simulink model "LithiumIonSieve"  (R2025b)
settings: Solver=VariableStepAuto  StartTime=0.0  StopTime=3600*48  RelTol=1e-3
undefined symbols (not defined in the file or in its folder): t_clean, t_regen, t_service
libraries: fl_lib x19, customization_lib x14, nesl_utility x1
settings Model: Creator=ndegoede  LastModifiedBy=degoede
settings SimscapeCC: SimscapeLogType=all  SimscapeLogOpenViewer=on

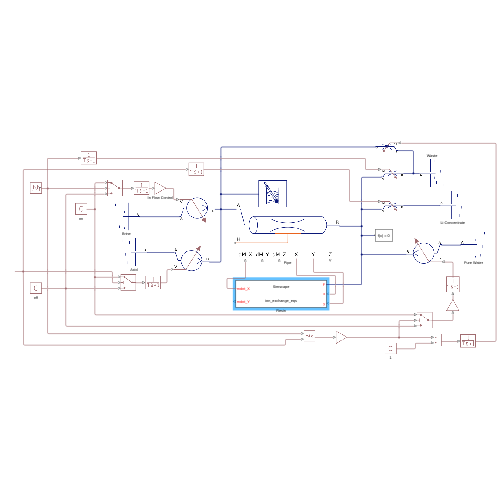
[thumbnail: Simulink's stored preview of the top-level diagram]
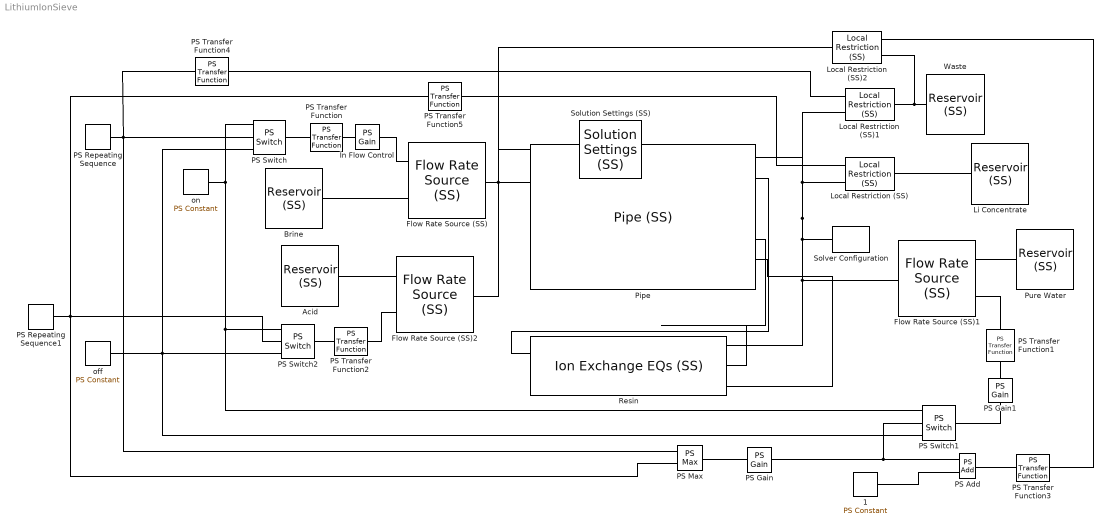
== system LithiumIonSieve ==
  1 : fl_lib/Physical Signals/Sources/PS Constant  constant=1
  Acid : customization_lib/solution/elements/Reservoir (SS)  pressure_spec=foundation.enum.pressure_spec.atmospheric  reservoir_pressure=0.101325 MPa  reservoir_temperature=293.15 K  reservoir_concentration=0 kg/m^3  reservoir_concentration_y=2e-4 g/l  reservoir_concentration_z=0 kg/m^3  area=0.01 m^2  custom_ports=false  length_A=1e-3 m
      settings: SourceProductName=Customization  InternalSimscapePortConfiguration="{\"Bottom\":[],\"Left\":[{\"id\":\"A\",\"label\":\"A\",\"type\":\"customization.solution.solution\"}],\"Right\":[],\"Top\":[]}"
  Brine : customization_lib/solution/elements/Reservoir (SS)  pressure_spec=foundation.enum.pressure_spec.atmospheric  reservoir_pressure=0.101325 MPa  reservoir_temperature=293.15 K  reservoir_concentration=1630 mg/l  reservoir_concentration_y=10^-6.5 g/l  reservoir_concentration_z=29000 mg/l  area=0.01 m^2  custom_ports=false  length_A=1e-3 m
      settings: SourceProductName=Customization  InternalSimscapePortConfiguration="{\"Bottom\":[],\"Left\":[{\"id\":\"A\",\"label\":\"A\",\"type\":\"customization.solution.solution\"}],\"Right\":[],\"Top\":[]}"
  Flow Rate Source (SS) : customization_lib/solution/sources/Flow Rate Source (SS)  source_type=foundation.enum.constant_controlled.controlled  flow_type=foundation.enum.mass_volumetric_flow.volumetric  mass_flow=0 kg/s  volumetric_flow=0 m^3/s  power_spec=foundation.enum.power_spec.isentropic  area=0.01 m^2  custom_ports=false  length_A=1e-3 m  length_B=1e-3 m
      settings: SourceProductName=Customization  InternalSimscapePortConfiguration="{\"Bottom\":[],\"Left\":[{\"id\":\"A\",\"label\":\"A\",\"type\":\"customization.solution.solution\"},{\"id\":\"V\",\"label\":\"V\",\"type\":\"input\"}],\"Right\":[{\"id\":\"B\",\"label\":\"B\",\"type\":\"customization.solution.solution\"}],\"Top\":[]}"
  Flow Rate Source (SS)1 : customization_lib/solution/sources/Flow Rate Source (SS)  source_type=foundation.enum.constant_controlled.controlled  flow_type=foundation.enum.mass_volumetric_flow.volumetric  mass_flow=0 kg/s  volumetric_flow=0 m^3/s  power_spec=foundation.enum.power_spec.isentropic  area=0.01 m^2  custom_ports=false  length_A=1e-3 m  length_B=1e-3 m
      settings: SourceProductName=Customization  InternalSimscapePortConfiguration="{\"Bottom\":[],\"Left\":[{\"id\":\"A\",\"label\":\"A\",\"type\":\"customization.solution.solution\"},{\"id\":\"V\",\"label\":\"V\",\"type\":\"input\"}],\"Right\":[{\"id\":\"B\",\"label\":\"B\",\"type\":\"customization.solution.solution\"}],\"Top\":[]}"
  Flow Rate Source (SS)2 : customization_lib/solution/sources/Flow Rate Source (SS)  source_type=foundation.enum.constant_controlled.controlled  flow_type=foundation.enum.mass_volumetric_flow.volumetric  mass_flow=0 kg/s  volumetric_flow=0 m^3/s  power_spec=foundation.enum.power_spec.isentropic  area=0.01 m^2  custom_ports=false  length_A=1e-3 m  length_B=1e-3 m
      settings: SourceProductName=Customization  InternalSimscapePortConfiguration="{\"Bottom\":[],\"Left\":[{\"id\":\"A\",\"label\":\"A\",\"type\":\"customization.solution.solution\"},{\"id\":\"V\",\"label\":\"V\",\"type\":\"input\"}],\"Right\":[{\"id\":\"B\",\"label\":\"B\",\"type\":\"customization.solution.solution\"}],\"Top\":[]}"
  In Flow Control : fl_lib/Physical Signals/Functions/PS Gain  gain=2
  Li Concentrate : customization_lib/solution/elements/Reservoir (SS)  pressure_spec=foundation.enum.pressure_spec.atmospheric  reservoir_pressure=0.101325 MPa  reservoir_temperature=293.15 K  reservoir_concentration=0 kg/m^3  reservoir_concentration_y=0 kg/m^3  reservoir_concentration_z=0 kg/m^3  area=0.01 m^2  custom_ports=false  length_A=1e-3 m
      settings: SourceProductName=Customization  InternalSimscapePortConfiguration="{\"Bottom\":[],\"Left\":[{\"id\":\"A\",\"label\":\"A\",\"type\":\"customization.solution.solution\"}],\"Right\":[],\"Top\":[]}"
  Local Restriction (SS) : customization_lib/solution/elements/Local Restriction (SS)  restriction_type=foundation.enum.restriction_type.variable  restriction_area=0.001 m^2  min_area=1e-5 m^2  max_area=0.005 m^2  area=0.01 m^2  Cd=0.64  Re_c=150  pressure_recovery=simscape.enum.onoff.on  custom_ports=false  length_A=1e-3 m  length_B=1e-3 m
      settings: SourceProductName=Customization  InternalSimscapePortConfiguration="{\"Bottom\":[],\"Left\":[{\"id\":\"A\",\"label\":\"A\",\"type\":\"customization.solution.solution\"},{\"id\":\"area_in\",\"label\":\"AR\",\"type\":\"input\"}],\"Right\":[{\"id\":\"B\",\"label\":\"B\",\"type\":\"customization.solution.solution\"}],\"Top\":[]}"
  Local Restriction (SS)1 : customization_lib/solution/elements/Local Restriction (SS)  restriction_type=foundation.enum.restriction_type.variable  restriction_area=0.001 m^2  min_area=1e-5 m^2  max_area=0.005 m^2  area=0.01 m^2  Cd=0.64  Re_c=150  pressure_recovery=simscape.enum.onoff.on  custom_ports=false  length_A=1e-3 m  length_B=1e-3 m
      settings: SourceProductName=Customization  InternalSimscapePortConfiguration="{\"Bottom\":[],\"Left\":[{\"id\":\"A\",\"label\":\"A\",\"type\":\"customization.solution.solution\"},{\"id\":\"area_in\",\"label\":\"AR\",\"type\":\"input\"}],\"Right\":[{\"id\":\"B\",\"label\":\"B\",\"type\":\"customization.solution.solution\"}],\"Top\":[]}"
  Local Restriction (SS)2 : customization_lib/solution/elements/Local Restriction (SS)  restriction_type=foundation.enum.restriction_type.variable  restriction_area=0.001 m^2  min_area=1e-5 m^2  max_area=0.005 m^2  area=0.01 m^2  Cd=0.64  Re_c=150  pressure_recovery=simscape.enum.onoff.on  custom_ports=false  length_A=1e-3 m  length_B=1e-3 m
      settings: SourceProductName=Customization  InternalSimscapePortConfiguration="{\"Bottom\":[],\"Left\":[{\"id\":\"A\",\"label\":\"A\",\"type\":\"customization.solution.solution\"},{\"id\":\"area_in\",\"label\":\"AR\",\"type\":\"input\"}],\"Right\":[{\"id\":\"B\",\"label\":\"B\",\"type\":\"customization.solution.solution\"}],\"Top\":[]}"
  PS Add : fl_lib/Physical Signals/Functions/PS Add
  PS Gain : fl_lib/Physical Signals/Functions/PS Gain  gain=-1
  PS Gain1 : fl_lib/Physical Signals/Functions/PS Gain  gain=2
  PS Max : fl_lib/Physical Signals/Nonlinear Operators/PS Max  ZeroCross=true
      settings: InternalSimscapePortConfiguration="{\"Bottom\":[],\"Left\":[{\"id\":\"I1\",\"label\":\"\",\"type\":\"input\"},{\"id\":\"I2\",\"label\":\"\",\"type\":\"input\"}],\"Right\":[{\"id\":\"O\",\"label\":\"\",\"type\":\"output\"}],\"Top\":[]}"
  PS Repeating Sequence : fl_lib/Physical Signals/Sources/PS Repeating Sequence  y_init=0  offset=0 s  sig_type=foundation.enum.SequenceSignalType.Discrete  durations=[t_service, t_clean, t_regen, t_clean] s  y_start=[1,0,0,0]  y_end=[1,0,0,0]
      settings: InternalSimscapePortConfiguration="{\"Bottom\":[],\"Left\":[],\"Right\":[{\"id\":\"Y\",\"label\":\"Y\",\"type\":\"output\"}],\"Top\":[]}"
  PS Repeating Sequence1 : fl_lib/Physical Signals/Sources/PS Repeating Sequence  y_init=0  offset=0 s  sig_type=foundation.enum.SequenceSignalType.Discrete  durations=[t_service, t_clean, t_regen, t_clean] s  y_start=[0,0,1,0]  y_end=[1,0,0,0]
      settings: InternalSimscapePortConfiguration="{\"Bottom\":[],\"Left\":[],\"Right\":[{\"id\":\"Y\",\"label\":\"Y\",\"type\":\"output\"}],\"Top\":[]}"
  PS Switch : fl_lib/Physical Signals/Nonlinear Operators/PS Switch  Threshold=0.5  ZeroCross=true
      settings: InternalSimscapePortConfiguration="{\"Bottom\":[],\"Left\":[{\"id\":\"I1\",\"label\":\"\",\"type\":\"input\"},{\"id\":\"I2\",\"label\":\"\",\"type\":\"input\"},{\"id\":\"I3\",\"label\":\"\",\"type\":\"input\"}],\"Right\":[{\"id\":\"O\",\"label\":\"\",\"type\":\"output\"}],\"Top\":[]}"
  PS Switch1 : fl_lib/Physical Signals/Nonlinear Operators/PS Switch  Threshold=-0.5  ZeroCross=true
      settings: InternalSimscapePortConfiguration="{\"Bottom\":[],\"Left\":[{\"id\":\"I1\",\"label\":\"\",\"type\":\"input\"},{\"id\":\"I2\",\"label\":\"\",\"type\":\"input\"},{\"id\":\"I3\",\"label\":\"\",\"type\":\"input\"}],\"Right\":[{\"id\":\"O\",\"label\":\"\",\"type\":\"output\"}],\"Top\":[]}"
  PS Switch2 : fl_lib/Physical Signals/Nonlinear Operators/PS Switch  Threshold=0.5  ZeroCross=true
      settings: InternalSimscapePortConfiguration="{\"Bottom\":[],\"Left\":[{\"id\":\"I1\",\"label\":\"\",\"type\":\"input\"},{\"id\":\"I2\",\"label\":\"\",\"type\":\"input\"},{\"id\":\"I3\",\"label\":\"\",\"type\":\"input\"}],\"Right\":[{\"id\":\"O\",\"label\":\"\",\"type\":\"output\"}],\"Top\":[]}"
  PS Transfer Function : fl_lib/Physical Signals/Linear Operators/PS Transfer Function  transfer_function_type=foundation.enum.transfer_function_type.lag  T=20 s  T1=2 s  T2=1 s  reset_method=foundation.enum.IntegratorResetSpec.None  initial_condition_spec=foundation.enum.IntegratorICSpec.Internal  y0=0 l/s
      settings: InternalSimscapePortConfiguration="{\"Bottom\":[],\"Left\":[{\"id\":\"U\",\"label\":\"\",\"type\":\"input\"}],\"Right\":[{\"id\":\"Y\",\"label\":\"\",\"type\":\"output\"}],\"Top\":[]}"
  PS Transfer Function1 : fl_lib/Physical Signals/Linear Operators/PS Transfer Function  transfer_function_type=foundation.enum.transfer_function_type.lag  T=20 s  T1=2 s  T2=1 s  reset_method=foundation.enum.IntegratorResetSpec.None  initial_condition_spec=foundation.enum.IntegratorICSpec.Internal  y0=0 l/s
      settings: InternalSimscapePortConfiguration="{\"Bottom\":[],\"Left\":[{\"id\":\"U\",\"label\":\"\",\"type\":\"input\"}],\"Right\":[{\"id\":\"Y\",\"label\":\"\",\"type\":\"output\"}],\"Top\":[]}"
  PS Transfer Function2 : fl_lib/Physical Signals/Linear Operators/PS Transfer Function  transfer_function_type=foundation.enum.transfer_function_type.lag  T=20 s  T1=2 s  T2=1 s  reset_method=foundation.enum.IntegratorResetSpec.None  initial_condition_spec=foundation.enum.IntegratorICSpec.Internal  y0=0 l/s
      settings: InternalSimscapePortConfiguration="{\"Bottom\":[],\"Left\":[{\"id\":\"U\",\"label\":\"\",\"type\":\"input\"}],\"Right\":[{\"id\":\"Y\",\"label\":\"\",\"type\":\"output\"}],\"Top\":[]}"
  PS Transfer Function3 : fl_lib/Physical Signals/Linear Operators/PS Transfer Function  transfer_function_type=foundation.enum.transfer_function_type.lag  T=20 s  T1=2 s  T2=1 s  reset_method=foundation.enum.IntegratorResetSpec.None  initial_condition_spec=foundation.enum.IntegratorICSpec.Internal  y0=0
      settings: InternalSimscapePortConfiguration="{\"Bottom\":[],\"Left\":[{\"id\":\"U\",\"label\":\"\",\"type\":\"input\"}],\"Right\":[{\"id\":\"Y\",\"label\":\"\",\"type\":\"output\"}],\"Top\":[]}"
  PS Transfer Function4 : fl_lib/Physical Signals/Linear Operators/PS Transfer Function  transfer_function_type=foundation.enum.transfer_function_type.lag  T=20 s  T1=2 s  T2=1 s  reset_method=foundation.enum.IntegratorResetSpec.None  initial_condition_spec=foundation.enum.IntegratorICSpec.Internal  y0=1
      settings: InternalSimscapePortConfiguration="{\"Bottom\":[],\"Left\":[{\"id\":\"U\",\"label\":\"\",\"type\":\"input\"}],\"Right\":[{\"id\":\"Y\",\"label\":\"\",\"type\":\"output\"}],\"Top\":[]}"
  PS Transfer Function5 : fl_lib/Physical Signals/Linear Operators/PS Transfer Function  transfer_function_type=foundation.enum.transfer_function_type.lag  T=20 s  T1=2 s  T2=1 s  reset_method=foundation.enum.IntegratorResetSpec.None  initial_condition_spec=foundation.enum.IntegratorICSpec.Internal  y0=0
      settings: InternalSimscapePortConfiguration="{\"Bottom\":[],\"Left\":[{\"id\":\"U\",\"label\":\"\",\"type\":\"input\"}],\"Right\":[{\"id\":\"Y\",\"label\":\"\",\"type\":\"output\"}],\"Top\":[]}"
  Pipe : customization_lib/solution/elements/Pipe (SS)  length=1 m  area=pi*0.1^2 m^2  Dh=0.2 m  Re_min=0.1  length_add=1 m  roughness=15e-6 m  Re_lam=2000  Re_tur=4000  shape_factor=64  Nu_lam=3.66  dynamic_compressibility=true  dM_X_source=true  dM_Y_source=true  dM_Z_source=true  dM_W_source=false  phi_source=false  inertia=false  p0=0.101325 MPa  T0=293.15 K  x0=0 kg/m^3  y0=0 kg/m^3  z0=0 kg/m^3  mdot0=0 kg/s  m_measure=false  p_measure=false  t_measure=false  pi_measure=false  x_measure=true  y_measure=true  z_measure=true  internal_concentration_gradient=false  flux_area=7.4 m^2  custom_ports=false  length_A=1e-3 m  length_B=1e-3 m
      settings: SourceProductName=Customization  InternalSimscapePortConfiguration="{\"Bottom\":[{\"id\":\"dM_X\",\"label\":\"dM_X\",\"type\":\"input\"},{\"id\":\"dM_Y\",\"label\":\"dM_Y\",\"type\":\"input\"},{\"id\":\"dM_Z\",\"label\":\"dM_Z\",\"type\":\"input\"},{\"id\":\"X\",\"label\":\"X\",\"type\":\"output\"},{\"id\":\"Y\",\"label\":\"Y\",\"type\":\"output\"},{\"id\":\"Z\",\"label\":\"Z\",\"type\":\"output\"}],\"Left\":[{\"id\":\"A\",\"label\":\"A\",\"type\":\"customization.solution.solution\"},{\"id\":\"H\",\"label\":\"H\",\"type\":\"foundation.thermal.thermal\"}],\"Right\":[{\"id\":\"B\",\"label\":\"B\",\"type\":\"customization.solution.solution\"}],\"Top\":[]}"
  Pure Water : customization_lib/solution/elements/Reservoir (SS)  pressure_spec=foundation.enum.pressure_spec.atmospheric  reservoir_pressure=0.101325 MPa  reservoir_temperature=293.15 K  reservoir_concentration=0 kg/m^3  reservoir_concentration_y=0 kg/m^3  reservoir_concentration_z=0 kg/m^3  area=0.01 m^2  custom_ports=false  length_A=1e-3 m
      settings: SourceProductName=Customization  InternalSimscapePortConfiguration="{\"Bottom\":[],\"Left\":[{\"id\":\"A\",\"label\":\"A\",\"type\":\"customization.solution.solution\"}],\"Right\":[],\"Top\":[]}"
  Resin : customization_lib/ion_exchange/Ion Exchange EQs (SS)  include_x=true  include_y=true  include_z=false  q_max=pi*0.1^2*4.7*3300*0.3 mol  k_spec=customization.ion_exchange.k_spec_options.k_x  k_x=2.5e-6/(4.7*0.2e-3) l/(mol*s)  k_y=1 l/s  k_z=1 l/(mol*s)  K_xy=2.8530e-5  K_xz=300  K_yx=1  K_yz=1  K_zx=1  K_zy=1  theta_x0=0  theta_y0=1
      settings: SourceProductName=Customization  InternalSimscapePortConfiguration="{\"Bottom\":[],\"Left\":[{\"id\":\"F\",\"label\":\"F\",\"type\":\"customization.solution.solution\"},{\"id\":\"x\",\"label\":\"x\",\"type\":\"input\"},{\"id\":\"y\",\"label\":\"y\",\"type\":\"input\"}],\"Right\":[{\"id\":\"mdot_x\",\"label\":\"mdot_X\",\"type\":\"output\"},{\"id\":\"mdot_y\",\"label\":\"mdot_Y\",\"type\":\"output\"}],\"Top\":[]}"
  Solution Settings (SS) : customization_lib/solution/utilities/Solution Settings (SS)  table_dimensions=foundation.enum.table_dimensions_TL.two_dimensional  T_TLU=[273.1600 : 10 : 373.16]' K  p_TLU=[0.01, 0.1, 5 : 5 : 50] MPa  p_atm=0.101325 MPa  pT_region_flag=foundation.enum.pT_region_TL.min_max  T_min=273.16 K  T_max=373.16 K  p_min=0.01 MPa  p_max=50 MPa  T_min_1D=273.16 K  T_max_1D=373.16 K  p_min_1D=0.01 MPa  p_max_1D=50 MPa  pT_validity_TLU=[1, 1, 1, 1, 1, 1, 1, 1, 1, 1, 1, 1; 1, 1, 1, 1, 1, 1, 1, 1, 1, 1, 1, 1; 1, 1, 1, 1, 1, 1, 1, 1, 1, 1, 1, 1; 1, 1, 1, 1, 1, 1, 1, 1, 1, 1, 1, 1; 1, 1, 1, 1, 1, 1, 1, 1, 1, 1, 1, 1; 0, 1, 1, 1, 1, 1, 1, 1, 1, 1, 1, 1; 0, 1, 1, 1, 1, 1, 1, 1, 1, 1, 1, 1; 0, 1, 1, 1, 1, 1, 1, 1, 1, 1, 1, 1; 0, 1, 1, 1, 1, 1, 1, 1, 1, 1, 1, 1; 0, 1, 1, 1, 1, 1, 1, 1, 1, 1, 1, 1; 0, 0, 1, 1, 1, 1, 1, 1, 1, 1, 1, 1]  properties_range_check=simscape.enum.assert.action.error  rho_parameterization_2D=foundation.enum.rho_parameterization_2D.rho_beta_alpha  rho_parameterization_1D=foundation.enum.rho_parameterization_1D.rho_vector  rho_TLU=[999.7973, 999.8431, 1002.3216, 1004.8218, 1007.293, 1009.7358, 1012.1506, 1014.5379, 1016.8979, 1019.2311, 1021.538, 1023.8188; 999.6579, 999.7009, 1002.0303, 1004.382, 1006.7084, 1009.0101, 1011.2874, 1013.5407, 1015.7703, 1017.9766, 1020.1599, 1022.3206; 998.1632, 998.2045, 1000.4375, 1002.6924, 1004.9239, 1007.1324, 1009.3183, 1011.4819, 1013.6236, 1015.7438, 1017.8428, 1019.921; 995.6057, 995.6458, 997.8186, 1000.0128, 1002.1841, 1004.3332, 1006.4603, 1008.566, 1010.6505, 1012.7144, 1014.758, 1016.7815; 992.1724, 992.2119, 994.3513, 996.5113, 998.6484, 1000.7633, 1002.8563, 1004.928, 1006.9788, 1009.009, 1011.0192, 1013.0097; 988.02, 988.0299, 990.1568, 992.3035, 994.4268, 996.5273, 998.6056, 1000.6622, 1002.6976, 1004.7123, 1006.7067, 1008.6813; 983.18, 983.1901, 985.3217, 987.4721, 989.5983, 991.7008, 993.7803, 995.8374, 997.8726, 999.8864, 1001.8795, 1003.8522; 977.75, 977.7583, 979.9094, 982.0783, 984.2216, 986.34, 988.4343, 990.505, 992.5529, 994.5786, 996.5825, 998.5654; 971.77, 971.7836, 973.9673, 976.1678, 978.3409, 980.4876, 982.6087, 984.7049, 986.7768, 988.8254, 990.8511, 992.8545; 965.26, 965.3023, 967.5311, 969.7753, 971.9901, 974.1764, 976.3354, 978.4676, 980.5741, 982.6556, 984.7129, 986.7465; 958.62, 958.6315, 960.627, 962.9267, 965.1944, 967.4314, 969.6387, 971.8173, 973.9681, 976.0921, 978.19, 980.2628] kg/m^3  beta_TLU=[1.9649, 1.9654, 1.9929, 2.0213, 2.0499, 2.0787, 2.1078, 2.1372, 2.1668, 2.1966, 2.2268, 2.2572; 2.0913, 2.0918, 2.1191, 2.1471, 2.1752, 2.2036, 2.2322, 2.261, 2.2899, 2.3191, 2.3485, 2.3781; 2.1786, 2.1791, 2.2067, 2.235, 2.2634, 2.2919, 2.3206, 2.3494, 2.3784, 2.4075, 2.4367, 2.4661; 2.2332, 2.2337, 2.2619, 2.2908, 2.3197, 2.3487, 2.3778, 2.407, 2.4363, 2.4657, 2.4951, 2.5246; 2.26, 2.2605, 2.2895, 2.3191, 2.3487, 2.3784, 2.4081, 2.4378, 2.4675, 2.4973, 2.5272, 2.5571; 2.2638, 2.2638, 2.2936, 2.324, 2.3544, 2.3848, 2.4151, 2.4455, 2.4758, 2.5062, 2.5365, 2.5669; 2.2472, 2.2472, 2.2779, 2.3092, 2.3403, 2.3715, 2.4025, 2.4336, 2.4646, 2.4955, 2.5264, 2.5573; 2.214, 2.214, 2.2455, 2.2776, 2.3096, 2.3415, 2.3733, 2.405, 2.4367, 2.4683, 2.4998, 2.5313; 2.1668, 2.1668, 2.1992, 2.2321, 2.2649, 2.2976, 2.3301, 2.3626, 2.3949, 2.4272, 2.4593, 2.4914; 2.1081, 2.1081, 2.1413, 2.175, 2.2086, 2.2421, 2.2754, 2.3085, 2.3415, 2.3744, 2.4072, 2.4399; 2.0494, 2.0494, 2.0739, 2.1084, 2.1428, 2.177, 2.211, 2.2449, 2.2786, 2.3121, 2.3455, 2.3788] GPa  alpha_TLU=1e-4 * [-.679, -.676, -.49, -.307, -.13, .041, .206, .365, .519, .668, .811, .949; .878, .881, .998, 1.114, 1.227, 1.337, 1.445, 1.549, 1.651, 1.75, 1.846, 1.939; 2.068, 2.069, 2.141, 2.213, 2.283, 2.352, 2.42, 2.486, 2.551, 2.614, 2.676, 2.736; 3.034, 3.035, 3.074, 3.113, 3.152, 3.191, 3.229, 3.267, 3.305, 3.341, 3.377, 3.413; 3.855, 3.856, 3.87, 3.884, 3.899, 3.914, 3.93, 3.946, 3.961, 3.977, 3.993, 4.009; 4.578, 4.578, 4.572, 4.566, 4.562, 4.558, 4.555, 4.552, 4.55, 4.549, 4.548, 4.547; 5.233, 5.233, 5.209, 5.186, 5.165, 5.144, 5.125, 5.107, 5.09, 5.074, 5.059, 5.045; 5.84, 5.84, 5.801, 5.762, 5.725, 5.691, 5.657, 5.625, 5.595, 5.566, 5.538, 5.512; 6.414, 6.414, 6.36, 6.307, 6.256, 6.208, 6.161, 6.117, 6.074, 6.033, 5.994, 5.956; 6.967, 6.967, 6.898, 6.831, 6.766, 6.705, 6.646, 6.589, 6.535, 6.482, 6.432, 6.384; 7.519, 7.519, 7.423, 7.342, 7.264, 7.189, 7.118, 7.049, 6.983, 6.92, 6.859, 6.8] 1/K  rho_TLU_2=[999.7973, 999.8431, 1002.3216, 1004.8218, 1007.293, 1009.7358, 1012.1506, 1014.5379, 1016.8979, 1019.2311, 1021.538, 1023.8188; 999.6579, 999.7009, 1002.0303, 1004.382, 1006.7084, 1009.0101, 1011.2874, 1013.5407, 1015.7703, 1017.9766, 1020.1599, 1022.3206; 998.1632, 998.2045, 1000.4375, 1002.6924, 1004.9239, 1007.1324, 1009.3183, 1011.4819, 1013.6236, 1015.7438, 1017.8428, 1019.921; 995.6057, 995.6458, 997.81864, 1000.0128, 1002.1841, 1004.3332, 1006.4603, 1008.566, 1010.6505, 1012.7144, 1014.758, 1016.7815; 992.1724, 992.2119, 994.3513, 996.5113, 998.6484, 1000.7633, 1002.8563, 1004.928, 1006.9788, 1009.009, 1011.0192, 1013.0097; 988.02, 988.0299, 990.1568, 992.3035, 994.4268, 996.5273, 998.6056, 1000.6622, 1002.6976, 1004.7123, 1006.7067, 1008.6813; 983.18, 983.1901, 985.3217, 987.4721, 989.5983, 991.7008, 993.7803, 995.8374, 997.8726, 999.8864, 1001.8795, 1003.8522; 977.75, 977.7583, 979.9094, 982.0783, 984.2216, 986.34, 988.4343, 990.505, 992.5529, 994.5786, 996.5825, 998.5654; 971.77, 971.7836, 973.9673, 976.1678, 978.3409, 980.4876, 982.6087, 984.7049, 986.7768, 988.8254, 990.8511, 992.8545; 965.26, 965.3023, 967.5311, 969.7753, 971.9901, 974.1764, 976.3354, 978.4676, 980.5741, 982.6556, 984.7129, 986.7465; 958.62, 958.6315, 960.627, 962.9267, 965.1944, 967.4314, 969.6387, 971.8173, 973.9681, 976.0921, 978.19, 980.2628] kg/m^3  rho_ref_3=998.21 kg/m^3  T_ref_3=293.16 K  p_ref_3=0.101325 MPa  beta_const_3=2.1791 GPa  alpha_const_3=2.0691e-4 1/K  rho_TLU_4=[999.84; 999.7; 998.2; 995.65; 992.21; 988.03; 983.19; 977.76; 971.78; 965.3; 958.8] kg/m^3  beta_const_4=2.1791 GPa  p_ref_4=0.101325 MPa  rho_ref_5=998.21 kg/m^3  T_ref_5=293.16 K  p_ref_5=0.101325 MPa  beta_const_5=2.1791 GPa  alpha_const_5=2.0691e-4 1/K  u_parameterization_2D=foundation.enum.u_parameterization_2D.u_cp  u_parameterization_1D=foundation.enum.u_parameterization_1D.u  u_TLU=[.0002, .0018, .086, .1588, .219, .267, .3034, .3288, .3436, .3483, .3435, .3294; 42.062, 42.06, 41.935, 41.804, 41.668, 41.527, 41.382, 41.233, 41.081, 40.924, 40.763, 40.599; 83.953, 83.948, 83.651, 83.349, 83.049, 82.749, 82.451, 82.153, 81.856, 81.56, 81.265, 80.971; 125.77, 125.76, 125.31, 124.86, 124.41, 123.97, 123.53, 123.1, 122.68, 122.25, 121.84, 121.42; 167.57, 167.56, 166.96, 166.37, 165.79, 165.21, 164.65, 164.09, 163.54, 163, 162.46, 161.94; 209.36, 209.36, 208.63, 207.9, 207.19, 206.48, 205.79, 205.11, 204.45, 203.79, 203.14, 202.5; 251.19, 251.19, 250.33, 249.47, 248.62, 247.79, 246.98, 246.18, 245.39, 244.62, 243.86, 243.12; 293.06, 293.06, 292.07, 291.07, 290.1, 289.14, 288.2, 287.28, 286.38, 285.49, 284.62, 283.77; 334.99, 334.99, 333.86, 332.73, 331.63, 330.54, 329.48, 328.44, 327.41, 326.41, 325.43, 324.46; 377, 377, 375.73, 374.46, 373.22, 372, 370.81, 369.64, 368.5, 367.38, 366.27, 365.19; 419.01, 419.01, 417.69, 416.27, 414.89, 413.54, 412.21, 410.91, 409.64, 408.4, 407.17, 405.98] kJ/kg  cp_TLU=[4.2199, 4.2194, 4.1957, 4.1726, 4.1508, 4.13, 4.1103, 4.0916, 4.0738, 4.0569, 4.0408, 4.0254; 4.1955, 4.1951, 4.1769, 4.1592, 4.1422, 4.1259, 4.1103, 4.0954, 4.0812, 4.0676, 4.0545, 4.0421; 4.1843, 4.184, 4.169, 4.1543, 4.1401, 4.1264, 4.1133, 4.1007, 4.0885, 4.0768, 4.0656, 4.0548; 4.1801, 4.1798, 4.1667, 4.1538, 4.1413, 4.1293, 4.1177, 4.1064, 4.0956, 4.0851, 4.075, 4.0653; 4.1796, 4.1794, 4.1675, 4.1558, 4.1444, 4.1334, 4.1227, 4.1123, 4.1023, 4.0926, 4.0832, 4.0741; 4.1813, 4.1813, 4.1702, 4.1592, 4.1484, 4.138, 4.1279, 4.1181, 4.1086, 4.0993, 4.0903, 4.0816; 4.185, 4.185, 4.1742, 4.1636, 4.1532, 4.1432, 4.1334, 4.1239, 4.1146, 4.1056, 4.0969, 4.0884; 4.1901, 4.1901, 4.1795, 4.169, 4.1588, 4.1489, 4.1393, 4.1299, 4.1207, 4.1118, 4.1032, 4.0947; 4.1968, 4.1968, 4.1862, 4.1757, 4.1655, 4.1555, 4.1458, 4.1364, 4.1273, 4.1183, 4.1096, 4.1012; 4.2052, 4.2052, 4.1944, 4.1837, 4.1733, 4.1632, 4.1534, 4.1438, 4.1345, 4.1255, 4.1166, 4.108; 4.2136, 4.2136, 4.2045, 4.1935, 4.1828, 4.1724, 4.1623, 4.1524, 4.1429, 4.1335, 4.1245, 4.1157] kJ/(K*kg)  u_TLU_2=[.0002, .0018, .086, .1588, .219, .267, .3034, .3288, .3436, .3483, .3435, .3294; 42.062, 42.06, 41.935, 41.804, 41.668, 41.527, 41.382, 41.233, 41.081, 40.924, 40.763, 40.599; 83.953, 83.948, 83.651, 83.349, 83.049, 82.749, 82.451, 82.153, 81.856, 81.56, 81.265, 80.971; 125.77, 125.76, 125.31, 124.86, 124.41, 123.97, 123.53, 123.1, 122.68, 122.25, 121.84, 121.42; 167.57, 167.56, 166.96, 166.37, 165.79, 165.21, 164.65, 164.09, 163.54, 163, 162.46, 161.94; 209.36, 209.36, 208.63, 207.9, 207.19, 206.48, 205.79, 205.11, 204.45, 203.79, 203.14, 202.5; 251.19, 251.19, 250.33, 249.47, 248.62, 247.79, 246.98, 246.18, 245.39, 244.62, 243.86, 243.12; 293.06, 293.06, 292.07, 291.07, 290.1, 289.14, 288.2, 287.28, 286.38, 285.49, 284.62, 283.77; 334.99, 334.99, 333.86, 332.73, 331.63, 330.54, 329.48, 328.44, 327.41, 326.41, 325.43, 324.46; 377, 377, 375.73, 374.46, 373.22, 372, 370.81, 369.64, 368.5, 367.38, 366.27, 365.19; 419.01, 419.01, 417.69, 416.27, 414.89, 413.54, 412.21, 410.91, 409.64, 408.4, 407.17, 405.98] kJ/kg  cp_TLU_3=[4.2199, 4.2194, 4.1957, 4.1726, 4.1508, 4.13, 4.1103, 4.0916, 4.0738, 4.0569, 4.0408, 4.0254; 4.1955, 4.1951, 4.1769, 4.1592, 4.1422, 4.1259, 4.1103, 4.0954, 4.0812, 4.0676, 4.0545, 4.0421; 4.1843, 4.184, 4.169, 4.1543, 4.1401, 4.1264, 4.1133, 4.1007, 4.0885, 4.0768, 4.0656, 4.0548; 4.1801, 4.1798, 4.1667, 4.1538, 4.1413, 4.1293, 4.1177, 4.1064, 4.0956, 4.0851, 4.075, 4.0653; 4.1796, 4.1794, 4.1675, 4.1558, 4.1444, 4.1334, 4.1227, 4.1123, 4.1023, 4.0926, 4.0832, 4.0741; 4.1813, 4.1813, 4.1702, 4.1592, 4.1484, 4.138, 4.1279, 4.1181, 4.1086, 4.0993, 4.0903, 4.0816; 4.185, 4.185, 4.1742, 4.1636, 4.1532, 4.1432, 4.1334, 4.1239, 4.1146, 4.1056, 4.0969, 4.0884; 4.1901, 4.1901, 4.1795, 4.169, 4.1588, 4.1489, 4.1393, 4.1299, 4.1207, 4.1118, 4.1032, 4.0947; 4.1968, 4.1968, 4.1862, 4.1757, 4.1655, 4.1555, 4.1458, 4.1364, 4.1273, 4.1183, 4.1096, 4.1012; 4.2052, 4.2052, 4.1944, 4.1837, 4.1733, 4.1632, 4.1534, 4.1438, 4.1345, 4.1255, 4.1166, 4.108; 4.2136, 4.2136, 4.2045, 4.1935, 4.1828, 4.1724, 4.1623, 4.1524, 4.1429, 4.1335, 4.1245, 4.1157] kJ/(K*kg)  u_TLU_4=[.0018; 42.06; 83.948; 125.76; 167.56; 209.36; 251.19; 293.06; 334.99; 377; 418.01] kJ/kg  cp_TLU_5=[4.2199; 4.1955; 4.1843; 4.1801; 4.1796; 4.1813; 4.185; 4.1901; 4.1968; 4.2052; 4.2136] kJ/(K*kg)  nu_TLU=[1.7917, 1.7914, 1.7763, 1.7615, 1.7473, 1.7338, 1.7208, 1.7085, 1.6967, 1.6854, 1.6747, 1.6645; 1.3061, 1.3059, 1.2986, 1.2914, 1.2845, 1.2779, 1.2716, 1.2656, 1.2598, 1.2543, 1.2491, 1.2441; 1.0032, 1.0032, .9995, .9959, .9924, .9891, .9859, .9829, .9801, .9774, .9748, .9724; .8006, .8005, .7987, .797, .7953, .7937, .7922, .7908, .7894, .7881, .787, .7859; .6577, .6577, .657, .6562, .6555, .6548, .6543, .6537, .6532, .6528, .6523, .652; .553, .553, .5529, .5527, .5526, .5525, .5524, .5524, .5524, .5524, .5524, .5525; .4739, .4739, .4741, .4743, .4745, .4747, .475, .4753, .4755, .4758, .4762, .4765; .4127, .4127, .4131, .4135, .4139, .4143, .4148, .4152, .4157, .4162, .4167, .4172; .3643, .3643, .3648, .3654, .3659, .3665, .367, .3676, .3682, .3688, .3694, .37; .3254, .3254, .3261, .3267, .3273, .328, .3286, .3293, .3299, .3306, .3312, .3319; .2866, .2866, .2945, .2952, .2959, .2965, .2972, .2979, .2986, .2993, .3, .3007] mm^2/s  nu_TLU_2=[1.7917; 1.3061; 1.0032; .8006; .6577; .553; .4739; .4127; .3643; .3254; .2866] mm^2/s  k_TLU=[561.04, 561.09, 563.8, 566.56, 569.32, 572.08, 574.82, 577.54, 580.24, 582.92, 585.57, 588.18; 580.02, 580.07, 582.45, 584.88, 587.32, 589.75, 592.18, 594.61, 597.02, 599.42, 601.8, 604.16; 598.44, 598.48, 600.73, 603.03, 605.33, 607.64, 609.94, 612.24, 614.54, 616.82, 619.1, 621.36; 615.48, 615.52, 617.73, 620, 622.26, 624.54, 626.81, 629.07, 631.34, 633.6, 635.85, 638.09; 630.6, 630.64, 632.87, 635.15, 637.44, 639.72, 642.01, 644.29, 646.57, 648.84, 651.11, 653.36; 643.61, 643.61, 645.88, 648.21, 650.53, 652.86, 655.18, 657.51, 659.82, 662.14, 664.44, 666.74; 654.39, 654.39, 656.73, 659.12, 661.5, 663.89, 666.27, 668.65, 671.02, 673.38, 675.74, 678.09; 663.13, 663.13, 665.54, 668, 670.46, 672.91, 675.36, 677.8, 680.24, 682.67, 685.09, 687.5; 670.02, 670.02, 672.51, 675.05, 677.59, 680.12, 682.64, 685.16, 687.67, 690.17, 692.66, 695.14; 675.27, 675.27, 677.85, 680.48, 683.11, 685.73, 688.34, 690.94, 693.53, 696.11, 698.68, 701.24; 680.52, 680.52, 681.77, 684.5, 687.22, 689.94, 692.64, 695.34, 698.02, 700.69, 703.35, 706] mW/(K*m)  k_TLU_2=[561.04; 580.02; 598.44; 615.48; 630.6; 643.61; 654.39; 663.13; 670.02; 675.27; 680.52] mW/(K*m)  D=0.875e-3 mm^2/s  rho_species=2000 kg/m^3  M=6.94 g/mol  i=1  R=8.314 J/(K*mol)  fm=0.62  nu_factor=2.5  D_y=0.875e-3 mm^2/s  rho_species_y=2000 kg/m^3  M_y=1 g/mol  i_y=1  D_z=0.875e-3 mm^2/s  rho_species_z=1.737 g/cm^3  M_z=24.3 g/mol  i_z=1
      settings: SourceProductName=Customization  InternalSimscapePortConfiguration="{\"Bottom\":[],\"Left\":[],\"Right\":[{\"id\":\"A\",\"label\":\"\",\"type\":\"customization.solution.solution\"}],\"Top\":[]}"
  Solver Configuration : nesl_utility/Solver Configuration  PhysicalDomain=network_engine_domain  SubClassName=solver  LeftPortType=input  RightPortType=generic  Tones=[]  Harmonics=[]  SimulateNoise=off  Profile=off  UseLocalSampling=off  EnableSwitchedLinearOptims=on  FrequencyDomain=off  UseCCode=off  RelTol=0.001  AbsTol=0.001  MinStep=1e-09  ToWorkspace=off  RevertToSquareIcSolve=off  NumHomotopyIterations=100  PhasorMode=off  PhasorModeNumHarmonics=1  ConsistencySolver=NEWTON_XTOL_AFTER_FTOL  IndexReductionMethod=DerivativeReplacement  DoDC=off  ResidualTolerance=1e-09  ConsistencyTolSource=GLOBAL  ConsistencyAbsTol=0.001  ConsistencyRelTol=0.001  ConsistencyTolFactor=0.001  UseLocalSolver=off  LocalSolverChoice=NE_BACKWARD_EULER_ADVANCER  ResolveIndetEquations=on  FunctionEvalNumThread=1  LocalSolverSampleTime=0.001  DoFixedCost=off  MaxNonlinIter=3  MaxModeIter=2  ComputeImpulses=off  ImpulseIterations=2  LinearAlgebra=auto  LinearAlgebraNumThread=0  EquationFormulation=NE_TIME_EF  DelaysMemoryBudget=1024  AutomaticFiltering=on  FilteringTimeConstant=0.001  PartitionStorageMethod=AS_NEEDED  PartitionMemoryBudget=1024  PartitionMethod=ROBUST  MultibodyUseLocalSolver=off  MultibodyLocalSolverChoice=ODE1  MultibodyLocalSolverSampleTime=0.001
  Waste : customization_lib/solution/elements/Reservoir (SS)  pressure_spec=foundation.enum.pressure_spec.atmospheric  reservoir_pressure=0.101325 MPa  reservoir_temperature=293.15 K  reservoir_concentration=0 kg/m^3  reservoir_concentration_y=0 kg/m^3  reservoir_concentration_z=0 kg/m^3  area=0.01 m^2  custom_ports=false  length_A=1e-3 m
      settings: SourceProductName=Customization  InternalSimscapePortConfiguration="{\"Bottom\":[],\"Left\":[{\"id\":\"A\",\"label\":\"A\",\"type\":\"customization.solution.solution\"}],\"Right\":[],\"Top\":[]}"
  off : fl_lib/Physical Signals/Sources/PS Constant  constant=0 l/s
  on : fl_lib/Physical Signals/Sources/PS Constant  constant=1 l/min
  connections:
  Resin/LConn1 -- Local Restriction (SS)1/LConn1 -- Local Restriction (SS)/LConn1 -- Pipe/RConn1 -- Solver Configuration/RConn1 -- Flow Rate Source (SS)1/RConn1
  Resin/LConn2 -- Pipe/RConn5
  Flow Rate Source (SS)/RConn1 -- Flow Rate Source (SS)2/RConn1 -- Local Restriction (SS)2/RConn1 -- Solution Settings (SS)/RConn1 -- Pipe/LConn1
  Brine/LConn1 -- Flow Rate Source (SS)/LConn1
  Flow Rate Source (SS)1/LConn1 -- Pure Water/LConn1
  Flow Rate Source (SS)2/LConn1 -- Acid/LConn1
  Flow Rate Source (SS)2/LConn2 -- PS Transfer Function2/RConn1
  Flow Rate Source (SS)/LConn2 -- In Flow Control/RConn1
  Flow Rate Source (SS)1/LConn2 -- PS Transfer Function1/RConn1
  off/RConn1 -- PS Switch/LConn3 -- PS Switch1/LConn3 -- PS Switch2/LConn3
  PS Switch/RConn1 -- PS Transfer Function/LConn1
  PS Switch1/RConn1 -- PS Gain1/LConn1
  PS Switch2/RConn1 -- PS Transfer Function2/LConn1
  on/RConn1 -- PS Switch2/LConn1 -- PS Switch1/LConn1 -- PS Switch/LConn1
  PS Max/LConn1 -- PS Transfer Function4/LConn1 -- PS Repeating Sequence/RConn1 -- PS Switch/LConn2
  PS Gain/LConn1 -- PS Max/RConn1
  PS Switch1/LConn2 -- PS Add/LConn1 -- PS Gain/RConn1
  Local Restriction (SS)1/RConn1 -- Local Restriction (SS)2/LConn1 -- Waste/LConn1
  Local Restriction (SS)/LConn2 -- PS Transfer Function5/RConn1
  Local Restriction (SS)/RConn1 -- Li Concentrate/LConn1
  PS Gain1/RConn1 -- PS Transfer Function1/LConn1
  Local Restriction (SS)2/LConn2 -- PS Transfer Function3/RConn1
  Local Restriction (SS)1/LConn2 -- PS Transfer Function4/RConn1
  PS Transfer Function5/LConn1 -- PS Max/LConn2 -- PS Switch2/LConn2 -- PS Repeating Sequence1/RConn1
  PS Add/RConn1 -- PS Transfer Function3/LConn1
  1/RConn1 -- PS Add/LConn2
  In Flow Control/LConn1 -- PS Transfer Function/RConn1
  Pipe/RConn6 -- Resin/LConn3
  Resin/RConn1 -- Pipe/RConn2
